simulink library "PacketizedNetworkLib"  (R2025b)
settings: Solver=VariableStepAuto  StartTime=0.0  StopTime=10.0  RelTol=1e-3
values from neighbouring files (symbols this model uses):
  dfeRef = [0.707106781187 -0.707106781187 0.707106781187 0.707106781187 -0.707106781187 0.707106781187 0.707106781187 0.707106781187 0.707106781187 0.707106781187 -0.707106781187 0.707106781187 ... (500 elements, 500x1)]    [networkParams.mat]
  L3payload = [0 0 0 1 0 0 0 0 1 1 1 0 ... (1040 elements, 1040x1)]    [networkParams.mat]
  ppdu_bb = [0 0 1 1 0 0 0 0 1 1 0 0 ... (2280 elements, 2280x1)]    [networkParams.mat]
  Ts = 1e-07    [networkParams.mat]
undefined symbols (not defined in the file or in its folder): AckDestAddre, DestAddre, dfilt, High, lambda, NodeAddre, pseed
libraries: $bdroot x19, hdlsllib x5, dspsigops x5, dspswit3 x3, simulink x3, dspindex x3, commdigbbndpm3 x2, simulink_extras x2, commfilt2 x2, commchan3 x1, dspmathops x1, dsparch4 x1
(part 2 of 3)

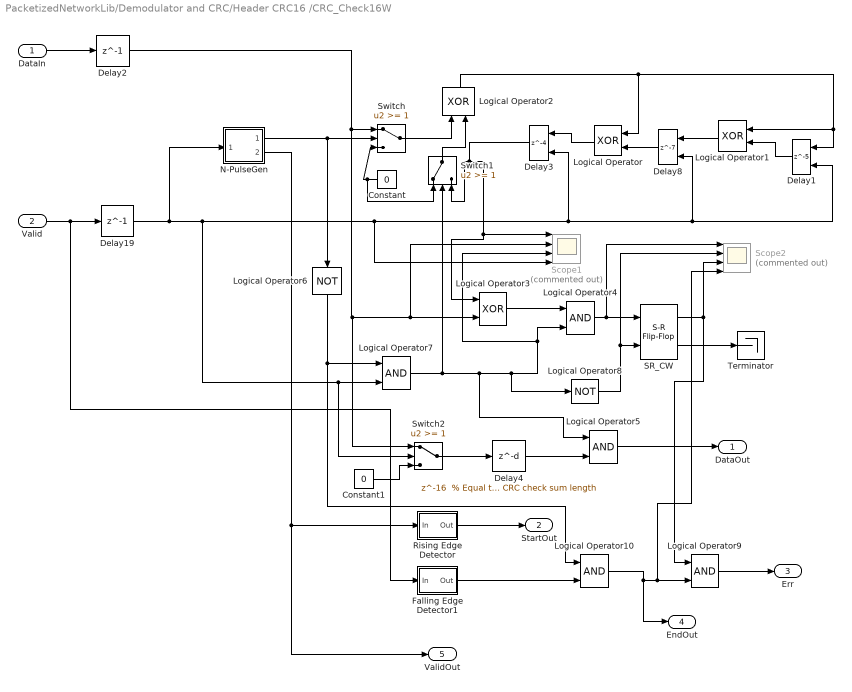
== system PacketizedNetworkLib/Demodulator and CRC/Header CRC16 /CRC_Check16W ==
  DataIn : Inport
  Valid : Inport  Port=2
  Constant : Constant  Value=0  OutDataTypeStr=boolean  SampleTime=-1
  Constant1 : Constant  Value=0  OutDataTypeStr=boolean  SampleTime=-1
  Delay1 : Delay  DelayLength=5  InitialCondition=0  ExternalReset=Rising
      settings: InputPortMap=u0,r5
  Delay19 : Delay  DelayLength=1
  Delay2 : Delay  DelayLength=1
  Delay3 : Delay  DelayLength=4  InitialCondition=0  ExternalReset=Rising
      settings: InputPortMap=u0,r5
  Delay4 : Delay  DelayLength="16  % Equal to the CRC check sum length"  InitialCondition=0
  Delay8 : Delay  DelayLength=7  InitialCondition=0  ExternalReset=Rising
      settings: InputPortMap=u0,r5
  Falling Edge Detector1 : Subsystem
  Logical Operator{,1..3} (4 alike) : Logic  Operator=XOR  AllPortsSameDT=off  OutDataTypeStr=boolean
  Logical Operator{4..5,7,9..10} (5 alike) : Logic  AllPortsSameDT=off  OutDataTypeStr=boolean
  Logical Operator6 : Logic  Operator=NOT  AllPortsSameDT=off  OutDataTypeStr=boolean
  Logical Operator8 : Logic  Operator=NOT  AllPortsSameDT=off  OutDataTypeStr=boolean
  N-PulseGen : Subsystem
  Rising Edge Detector : Subsystem
  SR_CW : simulink_extras/Flip Flops/S-R Flip-Flop  initial_condition=0
  Scope1 : Scope  Commented=on  NumInputPorts=4
      settings: ActiveDisplayYMinimum=-0.125  ActiveDisplayYMaximum=1.125  DataLoggingVariableName=ScopeData4  DataLoggingSaveFormat=Array
  Scope2 : Scope  Commented=on  NumInputPorts=4
      settings: ActiveDisplayYMinimum=-1  ActiveDisplayYMaximum=1  DataLoggingSaveFormat=Array
  Switch : Switch  Threshold=1  OutDataTypeStr=Inherit: Inherit via back propagation  SaturateOnIntegerOverflow=off
  Switch1 : Switch  Threshold=1  OutDataTypeStr=Inherit: Inherit via back propagation  SaturateOnIntegerOverflow=off
  Switch2 : Switch  Threshold=1  OutDataTypeStr=Inherit: Inherit via back propagation  SaturateOnIntegerOverflow=off
  Terminator : Terminator
  DataOut : Outport  VectorParamsAs1DForOutWhenUnconnected=off
  StartOut : Outport  Port=2  VectorParamsAs1DForOutWhenUnconnected=off
  Err : Outport  Port=3  VectorParamsAs1DForOutWhenUnconnected=off
  EndOut : Outport  Port=4  VectorParamsAs1DForOutWhenUnconnected=off
  ValidOut : Outport  Port=5  VectorParamsAs1DForOutWhenUnconnected=off
  wires:
  Logical Operator5/1 -> DataOut/1
  Logical Operator/1 -> Delay3/1
  Logical Operator10/1 -> Logical Operator9/2, Scope2/4, EndOut/1
  Delay19/1 -> N-PulseGen/1(In1), Switch2/2, Logical Operator7/2, Delay3/2, Delay1/2, Delay8/2, Scope1/4
  N-PulseGen/2(Out2) -> Rising Edge Detector/1(In), ValidOut/1
  Switch2/1 -> Delay4/1
  Constant1/1 -> Switch2/3
  Valid/1 -> Delay19/1, Falling Edge Detector1/1(In)
  Delay2/1 -> Logical Operator3/2, Scope1/2, Switch2/1, Switch/1
  Switch1/1 -> Logical Operator2/2
  Logical Operator6/1 -> Logical Operator7/1, Logical Operator10/1
  Delay1/1 -> Logical Operator1/2
  Logical Operator1/1 -> Delay8/1
  Delay8/1 -> Logical Operator/2
  Logical Operator8/1 -> Scope2/2, SR_CW/2
  Logical Operator7/1 -> Logical Operator4/2, Scope1/3, Logical Operator8/1, Logical Operator5/1, Switch1/2
  Logical Operator3/1 -> Logical Operator4/1
  N-PulseGen/1(Out1) -> Switch/2, Logical Operator6/1
  Logical Operator4/1 -> Scope2/1, SR_CW/1
  DataIn/1 -> Delay2/1
  Switch/1 -> Logical Operator2/1
  Delay3/1 -> Switch1/3, Scope1/1, Logical Operator3/1
  Constant/1 -> Switch/3, Switch1/1
  Logical Operator9/1 -> Err/1
  Falling Edge Detector1/1(Out) -> Logical Operator10/2
  SR_CW/1 -> Scope2/3, Logical Operator9/1
  Delay4/1 -> Logical Operator5/2
  Rising Edge Detector/1(Out) -> StartOut/1
  SR_CW/2 -> Terminator/1
  Logical Operator2/1 -> Logical Operator1/1, Delay1/1, Logical Operator/1

== system PacketizedNetworkLib/Demodulator and CRC/Pyld CRC32/Falling Edge Detector1 ==
  In : Inport
  Data Type Conversion2 : DataTypeConversion  OutDataTypeStr=boolean
  Delay : Delay  DelayLength=1  InitialCondition=1
  Logical Operator1 : Logic
  Logical Operator3 : Logic  Operator=NOT  Inputs=1
  Out : Outport  VectorParamsAs1DForOutWhenUnconnected=off
  wires:
  Logical Operator3/1 -> Logical Operator1/1
  Data Type Conversion2/1 -> Logical Operator3/1, Delay/1
  Delay/1 -> Logical Operator1/2
  In/1 -> Data Type Conversion2/1
  Logical Operator1/1 -> Out/1

== system PacketizedNetworkLib/Demodulator and CRC/Pyld CRC32/Rising Edge Detector ==
  In : Inport
  Data Type Conversion2 : DataTypeConversion  OutDataTypeStr=boolean
  Delay : Delay  DelayLength=1  InitialCondition=1
  Logical Operator : Logic  Operator=NOT  Inputs=1
  Logical Operator1 : Logic
  Out : Outport  VectorParamsAs1DForOutWhenUnconnected=off
  wires:
  Data Type Conversion2/1 -> Logical Operator1/1, Delay/1
  Logical Operator/1 -> Logical Operator1/2
  In/1 -> Data Type Conversion2/1
  Logical Operator1/1 -> Out/1
  Delay/1 -> Logical Operator/1

== system PacketizedNetworkLib/PHY//MAC Transceiver/Subsystem/BusSwitchFunIn ==
  Sel : Inport
  In1 : Inport  Port=2
  In2 : Inport  Port=3
  Bus Creator : BusCreator  Inputs=6
  Bus Selector1 : BusSelector  OutputSignals=TxDataFail,TxDataDone,TxDataOn,TxAckOn,BOTime,AckWaitTime
  Bus Selector2 : BusSelector  OutputSignals=TxDataFail,TxDataDone,TxDataOn,TxAckOn,BOTime,AckWaitTime
  Switch{,1..5} (6 alike) : Switch  Criteria=u2 > Threshold  SaturateOnIntegerOverflow=off  InputSameDT=off
  Out : Outport  VectorParamsAs1DForOutWhenUnconnected=off
  wires:
  Bus Creator/1 -> Out/1
  Switch5/1 -> Bus Creator/6
  Switch4/1 -> Bus Creator/5
  Switch3/1 -> Bus Creator/4
  Switch2/1 -> Bus Creator/3
  Switch1/1 -> Bus Creator/2
  Switch/1 -> Bus Creator/1
  In1/1 -> Bus Selector1/1
  Bus Selector1/6 -> Switch5/1  "<AckWaitTime>"
  Bus Selector1/5 -> Switch4/1  "<BOTime>"
  Bus Selector1/2 -> Switch1/1  "<TxDataDone>"
  Bus Selector1/1 -> Switch/1  "<TxDataFail>"
  Sel/1 -> Switch/2, Switch2/2, Switch5/2, Switch4/2, Switch3/2, Switch1/2
  Bus Selector1/3 -> Switch2/1  "<TxDataOn>"
  Bus Selector1/4 -> Switch3/1  "<TxAckOn>"
  Bus Selector2/1 -> Switch/3  "<TxDataFail>"
  Bus Selector2/2 -> Switch1/3  "<TxDataDone>"
  Bus Selector2/3 -> Switch2/3  "<TxDataOn>"
  Bus Selector2/4 -> Switch3/3  "<TxAckOn>"
  Bus Selector2/5 -> Switch4/3  "<BOTime>"
  Bus Selector2/6 -> Switch5/3  "<AckWaitTime>"
  In2/1 -> Bus Selector2/1

== system PacketizedNetworkLib/PHY//MAC Transceiver/Subsystem/BusSwitchFunOut ==
  Sel : Inport
  In : Inport  Port=2
  1to2_1 : Subsystem
  1to2_2 : Subsystem
  1to2_3 : Subsystem
  1to2_5 : Subsystem
  1to2_6 : Subsystem
  1to2_Integer : Subsystem
  Bus Creator1 : BusCreator  Inputs=6
  Bus Creator2 : BusCreator  Inputs=6
  Bus Selector1 : BusSelector  OutputSignals=TxLength,TxEn,signal3,signal4,signal5,signal6
  Out1 : Outport  VectorParamsAs1DForOutWhenUnconnected=off
  Out2 : Outport  Port=2  VectorParamsAs1DForOutWhenUnconnected=off
  wires:
  Bus Selector1/4 -> 1to2_3/1(In)  "<signal4>"
  Bus Selector1/3 -> 1to2_2/1(In)  "<signal3>"
  Bus Selector1/1 -> 1to2_Integer/1(In)  "<TxLength>"
  Bus Selector1/2 -> 1to2_1/1(In)  "<TxEn>"
  Bus Selector1/5 -> 1to2_5/1(In)  "<signal5>"
  Bus Selector1/6 -> 1to2_6/1(In)  "<signal6>"
  In/1 -> Bus Selector1/1
  Bus Creator2/1 -> Out1/1
  Bus Creator1/1 -> Out2/1
  Sel/1 -> 1to2_1/2(C), 1to2_2/2(C), 1to2_3/2(C), 1to2_6/2(C), 1to2_5/2(C), 1to2_Integer/2(C)
  1to2_Integer/1(Out1) -> Bus Creator2/1
  1to2_1/1(Out1) -> Bus Creator2/2
  1to2_2/1(Out1) -> Bus Creator2/3
  1to2_3/1(Out1) -> Bus Creator2/4
  1to2_5/1(Out1) -> Bus Creator2/5
  1to2_6/1(Out1) -> Bus Creator2/6
  1to2_Integer/2(Out2) -> Bus Creator1/1
  1to2_1/2(Out2) -> Bus Creator1/2
  1to2_2/2(Out2) -> Bus Creator1/3
  1to2_5/2(Out2) -> Bus Creator1/5
  1to2_3/2(Out2) -> Bus Creator1/4
  1to2_6/2(Out2) -> Bus Creator1/6

== system PacketizedNetworkLib/Receiver/DFE /DFE_Cell_FBW1 ==
  note: w(i)
  note: The Basic Cell of the Feedbackward Part of DFE Equalizer
      |
      | yd(i+1)= w(i+1).*d(i);
      | w(i+1)=w(i)+ m*D* w(i)=w(i)+etmu*conj(x(i));
      |
      | Note: All variables here are scalars
  note: w(i+1)
  d(i) : Inport
  etmu : Inport  Port=2
  " Unit_Delay1" : UnitDelay  SampleTime=-1  HasFrameUpgradeWarning=on
  " Unit_Delay2" : UnitDelay  SampleTime=-1  HasFrameUpgradeWarning=on
  Math Function : Math  Operator=conj  SignedPower=on
  Product1 : Product  InputSameDT=on  RndMeth=Zero  SaturateOnIntegerOverflow=on  OutDataTypeStr=Inherit: Same as first input
  Product2 : Product  InputSameDT=on  RndMeth=Zero  SaturateOnIntegerOverflow=on  OutDataTypeStr=Inherit: Same as first input
  Sum : Sum  InputSameDT=on  SaturateOnIntegerOverflow=on  OutDataTypeStr=Inherit: Same as first input
  "Unit_Delay1 " : UnitDelay  SampleTime=-1  HasFrameUpgradeWarning=on
  "d(i-1) " : Outport  VectorParamsAs1DForOutWhenUnconnected=off
  yd(i+1) : Outport  Port=2  VectorParamsAs1DForOutWhenUnconnected=off
  wires:
  " Unit_Delay1"/1 -> Product2/1
  Math Function/1 -> Product2/2
  d(i)/1 -> "Unit_Delay1 "/1, Product1/2
  etmu/1 -> " Unit_Delay1"/1
  "Unit_Delay1 "/1 -> "d(i-1) "/1, Math Function/1
  " Unit_Delay2"/1 -> Sum/1
  Sum/1 -> " Unit_Delay2"/1, Product1/1
  Product1/1 -> yd(i+1)/1
  Product2/1 -> Sum/2

== system PacketizedNetworkLib/Receiver/DFE /DFE_Cell_FBW2 ==
  note: w(i+1)
  note: The Basic Cell of the Feedbackward Part of DFE Equalizer
      |
      | yd(i+1)= w(i+1).*d(i);
      | w(i+1)=w(i)+ m*D* w(i)=w(i)+etmu*conj(x(i));
      |
      | Note: All variables here are scalars
  note: w(i)
  d(i) : Inport
  etmu : Inport  Port=2
  " Unit_Delay1" : UnitDelay  SampleTime=-1  HasFrameUpgradeWarning=on
  " Unit_Delay2" : UnitDelay  SampleTime=-1  HasFrameUpgradeWarning=on
  Math Function : Math  Operator=conj  SignedPower=on
  Product1 : Product  InputSameDT=on  RndMeth=Zero  SaturateOnIntegerOverflow=on  OutDataTypeStr=Inherit: Same as first input
  Product2 : Product  InputSameDT=on  RndMeth=Zero  SaturateOnIntegerOverflow=on  OutDataTypeStr=Inherit: Same as first input
  Sum : Sum  InputSameDT=on  SaturateOnIntegerOverflow=on  OutDataTypeStr=Inherit: Same as first input
  "Unit_Delay1 " : UnitDelay  SampleTime=-1  HasFrameUpgradeWarning=on
  "d(i-1) " : Outport  VectorParamsAs1DForOutWhenUnconnected=off
  yd(i+1) : Outport  Port=2  VectorParamsAs1DForOutWhenUnconnected=off
  wires:
  Product2/1 -> Sum/2
  Product1/1 -> yd(i+1)/1
  Sum/1 -> Product1/1, " Unit_Delay2"/1
  " Unit_Delay2"/1 -> Sum/1
  "Unit_Delay1 "/1 -> Math Function/1, "d(i-1) "/1
  etmu/1 -> " Unit_Delay1"/1
  d(i)/1 -> Product1/2, "Unit_Delay1 "/1
  Math Function/1 -> Product2/2
  " Unit_Delay1"/1 -> Product2/1

== system PacketizedNetworkLib/Receiver/DFE /DFE_Cell_FBW3 ==
  note: w(i+1)
  note: The Basic Cell of the Feedbackward Part of DFE Equalizer
      |
      | yd(i+1)= w(i+1).*d(i);
      | w(i+1)=w(i)+ m*D* w(i)=w(i)+etmu*conj(x(i));
      |
      | Note: All variables here are scalars
  note: w(i)
  d(i) : Inport
  etmu : Inport  Port=2
  " Unit_Delay1" : UnitDelay  SampleTime=-1  HasFrameUpgradeWarning=on
  " Unit_Delay2" : UnitDelay  SampleTime=-1  HasFrameUpgradeWarning=on
  Math Function : Math  Operator=conj  SignedPower=on
  Product1 : Product  InputSameDT=on  RndMeth=Zero  SaturateOnIntegerOverflow=on  OutDataTypeStr=Inherit: Same as first input
  Product2 : Product  InputSameDT=on  RndMeth=Zero  SaturateOnIntegerOverflow=on  OutDataTypeStr=Inherit: Same as first input
  Sum : Sum  InputSameDT=on  SaturateOnIntegerOverflow=on  OutDataTypeStr=Inherit: Same as first input
  "Unit_Delay1 " : UnitDelay  SampleTime=-1  HasFrameUpgradeWarning=on
  "d(i-1) " : Outport  VectorParamsAs1DForOutWhenUnconnected=off
  yd(i+1) : Outport  Port=2  VectorParamsAs1DForOutWhenUnconnected=off
  wires:
  Product2/1 -> Sum/2
  Product1/1 -> yd(i+1)/1
  Sum/1 -> " Unit_Delay2"/1, Product1/1
  " Unit_Delay2"/1 -> Sum/1
  "Unit_Delay1 "/1 -> Math Function/1, "d(i-1) "/1
  etmu/1 -> " Unit_Delay1"/1
  d(i)/1 -> Product1/2, "Unit_Delay1 "/1
  Math Function/1 -> Product2/2
  " Unit_Delay1"/1 -> Product2/1

== system PacketizedNetworkLib/Receiver/DFE /DFE_Cell_FBW4 ==
  note: w(i+1)
  note: The Basic Cell of the Feedbackward Part of DFE Equalizer
      |
      | yd(i+1)= w(i+1).*d(i);
      | w(i+1)=w(i)+ m*D* w(i)=w(i)+etmu*conj(x(i));
  note: w(i)
  note: DFE Equalizer
  d(i) : Inport
  etmu : Inport  Port=2
  " Unit_Delay1" : UnitDelay  SampleTime=-1  HasFrameUpgradeWarning=on
  " Unit_Delay2" : UnitDelay  SampleTime=-1  HasFrameUpgradeWarning=on
  Math Function : Math  Operator=conj  SignedPower=on
  Product1 : Product  InputSameDT=on  RndMeth=Zero  SaturateOnIntegerOverflow=on  OutDataTypeStr=Inherit: Same as first input
  Product2 : Product  InputSameDT=on  RndMeth=Zero  SaturateOnIntegerOverflow=on  OutDataTypeStr=Inherit: Same as first input
  Sum : Sum  InputSameDT=on  SaturateOnIntegerOverflow=on  OutDataTypeStr=Inherit: Same as first input
  "Unit_Delay1 " : UnitDelay  SampleTime=-1  HasFrameUpgradeWarning=on
  "d(i-1) " : Outport  VectorParamsAs1DForOutWhenUnconnected=off
  yd(i+1) : Outport  Port=2  VectorParamsAs1DForOutWhenUnconnected=off
  wires:
  Product2/1 -> Sum/2
  Product1/1 -> yd(i+1)/1
  Sum/1 -> " Unit_Delay2"/1, Product1/1
  " Unit_Delay2"/1 -> Sum/1
  "Unit_Delay1 "/1 -> "d(i-1) "/1, Math Function/1
  etmu/1 -> " Unit_Delay1"/1
  d(i)/1 -> Product1/2, "Unit_Delay1 "/1
  Math Function/1 -> Product2/2
  " Unit_Delay1"/1 -> Product2/1

== system PacketizedNetworkLib/Receiver/DFE /DFE_Cell_FBW5 ==
  note: w(i+1)
  note: The Basic Cell of the Feedbackward Part of DFE Equalizer
      |
      | yd(i+1)= w(i+1).*d(i);
      | w(i+1)=w(i)+ m*D* w(i)=w(i)+etmu*conj(x(i));
      |
      | Note: All variables here are scalars
  note: w(i)
  d(i) : Inport
  etmu : Inport  Port=2
  " Unit_Delay1" : UnitDelay  SampleTime=-1  HasFrameUpgradeWarning=on
  " Unit_Delay2" : UnitDelay  SampleTime=-1  HasFrameUpgradeWarning=on
  Math Function : Math  Operator=conj  SignedPower=on
  Product1 : Product  InputSameDT=on  RndMeth=Zero  SaturateOnIntegerOverflow=on  OutDataTypeStr=Inherit: Same as first input
  Product2 : Product  InputSameDT=on  RndMeth=Zero  SaturateOnIntegerOverflow=on  OutDataTypeStr=Inherit: Same as first input
  Sum : Sum  InputSameDT=on  SaturateOnIntegerOverflow=on  OutDataTypeStr=Inherit: Same as first input
  "Unit_Delay1 " : UnitDelay  SampleTime=-1  HasFrameUpgradeWarning=on
  "d(i-1) " : Outport  VectorParamsAs1DForOutWhenUnconnected=off
  yd(i+1) : Outport  Port=2  VectorParamsAs1DForOutWhenUnconnected=off
  wires:
  Product2/1 -> Sum/2
  Product1/1 -> yd(i+1)/1
  Sum/1 -> " Unit_Delay2"/1, Product1/1
  " Unit_Delay2"/1 -> Sum/1
  "Unit_Delay1 "/1 -> Math Function/1, "d(i-1) "/1
  etmu/1 -> " Unit_Delay1"/1
  d(i)/1 -> Product1/2, "Unit_Delay1 "/1
  Math Function/1 -> Product2/2
  " Unit_Delay1"/1 -> Product2/1

== system PacketizedNetworkLib/Receiver/DFE /DFE_Cell_FBW6 ==
  note: w(i+1)
  note: The Basic Cell of the Feedbackward Part of DFE Equalizer
      |
      | yd(i+1)= w(i+1).*d(i);
      | w(i+1)=w(i)+ m*D* w(i)=w(i)+etmu*conj(x(i));
      |
      | Note: All variables here are scalars
  note: w(i)
  d(i) : Inport
  etmu : Inport  Port=2
  " Unit_Delay1" : UnitDelay  SampleTime=-1  HasFrameUpgradeWarning=on
  " Unit_Delay2" : UnitDelay  SampleTime=-1  HasFrameUpgradeWarning=on
  Math Function : Math  Operator=conj  SignedPower=on
  Product1 : Product  InputSameDT=on  RndMeth=Zero  SaturateOnIntegerOverflow=on  OutDataTypeStr=Inherit: Same as first input
  Product2 : Product  InputSameDT=on  RndMeth=Zero  SaturateOnIntegerOverflow=on  OutDataTypeStr=Inherit: Same as first input
  Sum : Sum  InputSameDT=on  SaturateOnIntegerOverflow=on  OutDataTypeStr=Inherit: Same as first input
  "Unit_Delay1 " : UnitDelay  SampleTime=-1  HasFrameUpgradeWarning=on
  "d(i-1) " : Outport  VectorParamsAs1DForOutWhenUnconnected=off
  yd(i+1) : Outport  Port=2  VectorParamsAs1DForOutWhenUnconnected=off
  wires:
  Product2/1 -> Sum/2
  Product1/1 -> yd(i+1)/1
  Sum/1 -> Product1/1, " Unit_Delay2"/1
  " Unit_Delay2"/1 -> Sum/1
  "Unit_Delay1 "/1 -> "d(i-1) "/1, Math Function/1
  etmu/1 -> " Unit_Delay1"/1
  d(i)/1 -> Product1/2, "Unit_Delay1 "/1
  Math Function/1 -> Product2/2
  " Unit_Delay1"/1 -> Product2/1

== system PacketizedNetworkLib/Receiver/DFE /DFE_Cell_FFW1 ==
  note: w(i+1)
  note: The Basic Cell of the Feedforward Part of DFE Equalizer
      |
      | y(i+1)= ElimentSum (w(i+1).*x(i+1));
      | w(i+1)=w(i)+ m*D* w(i)=w(i)+etmu*conj(x(i));
      |
      | Note: y(+1) and etmu is a scalar, and x(i), w(i) are 2x1 vector. "2" is the decimation factor 2
  note: w(i)
  x(i+1) : Inport
  etmu : Inport  Port=2
  " Unit_Delay1" : UnitDelay  SampleTime=-1  HasFrameUpgradeWarning=on
  " Unit_Delay2" : UnitDelay  SampleTime=-1  HasFrameUpgradeWarning=on
  Math Function : Math  Operator=conj  SignedPower=on
  Product1 : Product  InputSameDT=on  RndMeth=Zero  SaturateOnIntegerOverflow=on  OutDataTypeStr=Inherit: Same as first input
  Product2 : Product  InputSameDT=on  RndMeth=Zero  SaturateOnIntegerOverflow=on  OutDataTypeStr=Inherit: Same as first input
  Sum : Sum  InputSameDT=on  SaturateOnIntegerOverflow=on  OutDataTypeStr=Inherit: Same as first input
  Sum of Elements : Sum  Inputs=+
  "Unit_Delay1 " : UnitDelay  SampleTime=-1  HasFrameUpgradeWarning=on
  "x(i) " : Outport  VectorParamsAs1DForOutWhenUnconnected=off
  y(i+1) : Outport  Port=2  VectorParamsAs1DForOutWhenUnconnected=off
  wires:
  Product2/1 -> Sum/2
  Product1/1 -> Sum of Elements/1
  " Unit_Delay2"/1 -> Sum/1
  "Unit_Delay1 "/1 -> Math Function/1, "x(i) "/1
  etmu/1 -> " Unit_Delay1"/1
  x(i+1)/1 -> Product1/2, "Unit_Delay1 "/1
  Math Function/1 -> Product2/2
  Sum of Elements/1 -> y(i+1)/1
  Sum/1 -> Product1/1, " Unit_Delay2"/1
  " Unit_Delay1"/1 -> Product2/1

== system PacketizedNetworkLib/Receiver/DFE /DFE_Cell_FFW2 ==
  note: w(i+1)
  note: The Basic Cell of the Feedforward Part of DFE Equalizer
      |
      | y(i+1)= ElimentSum (w(i+1).*x(i+1));
      | w(i+1)=w(i)+ m*D* w(i)=w(i)+etmu*conj(x(i));
      |
      | Note: y(+1) and etmu is a scalar, and x(i), w(i) are 2x1 vector. "2" is the decimation factor 2
  note: w(i)
  x(i+1) : Inport
  etmu : Inport  Port=2
  " Unit_Delay1" : UnitDelay  SampleTime=-1  HasFrameUpgradeWarning=on
  " Unit_Delay2" : UnitDelay  SampleTime=-1  HasFrameUpgradeWarning=on
  Math Function : Math  Operator=conj  SignedPower=on
  Product1 : Product  InputSameDT=on  RndMeth=Zero  SaturateOnIntegerOverflow=on  OutDataTypeStr=Inherit: Same as first input
  Product2 : Product  InputSameDT=on  RndMeth=Zero  SaturateOnIntegerOverflow=on  OutDataTypeStr=Inherit: Same as first input
  Sum : Sum  InputSameDT=on  SaturateOnIntegerOverflow=on  OutDataTypeStr=Inherit: Same as first input
  Sum of Elements : Sum  Inputs=+
  "Unit_Delay1 " : UnitDelay  SampleTime=-1  HasFrameUpgradeWarning=on
  "x(i) " : Outport  VectorParamsAs1DForOutWhenUnconnected=off
  y(i+1) : Outport  Port=2  VectorParamsAs1DForOutWhenUnconnected=off
  wires:
  Product2/1 -> Sum/2
  Product1/1 -> Sum of Elements/1
  " Unit_Delay2"/1 -> Sum/1
  "Unit_Delay1 "/1 -> Math Function/1, "x(i) "/1
  etmu/1 -> " Unit_Delay1"/1
  x(i+1)/1 -> Product1/2, "Unit_Delay1 "/1
  Math Function/1 -> Product2/2
  Sum of Elements/1 -> y(i+1)/1
  Sum/1 -> Product1/1, " Unit_Delay2"/1
  " Unit_Delay1"/1 -> Product2/1

== system PacketizedNetworkLib/Receiver/DFE /DFE_Cell_FFW3 ==
  note: w(i+1)
  note: The Basic Cell of the Feedforward Part of DFE Equalizer
      |
      | y(i+1)= ElimentSum (w(i+1).*x(i+1));
      | w(i+1)=w(i)+ m*D* w(i)=w(i)+etmu*conj(x(i));
      |
      | Note: y(+1) and etmu is a scalar, and x(i), w(i) are 2x1 vector. "2" is the decimation factor 2
  note: w(i)
  x(i+1) : Inport
  etmu : Inport  Port=2
  " Unit_Delay1" : UnitDelay  SampleTime=-1  HasFrameUpgradeWarning=on
  " Unit_Delay2" : UnitDelay  SampleTime=-1  HasFrameUpgradeWarning=on
  Math Function : Math  Operator=conj  SignedPower=on
  Product1 : Product  InputSameDT=on  RndMeth=Zero  SaturateOnIntegerOverflow=on  OutDataTypeStr=Inherit: Same as first input
  Product2 : Product  InputSameDT=on  RndMeth=Zero  SaturateOnIntegerOverflow=on  OutDataTypeStr=Inherit: Same as first input
  Sum : Sum  InputSameDT=on  SaturateOnIntegerOverflow=on  OutDataTypeStr=Inherit: Same as first input
  Sum of Elements : Sum  Inputs=+
  "Unit_Delay1 " : UnitDelay  SampleTime=-1  HasFrameUpgradeWarning=on
  "x(i) " : Outport  VectorParamsAs1DForOutWhenUnconnected=off
  y(i+1) : Outport  Port=2  VectorParamsAs1DForOutWhenUnconnected=off
  wires:
  Product2/1 -> Sum/2
  Product1/1 -> Sum of Elements/1
  " Unit_Delay2"/1 -> Sum/1
  "Unit_Delay1 "/1 -> Math Function/1, "x(i) "/1
  etmu/1 -> " Unit_Delay1"/1
  x(i+1)/1 -> Product1/2, "Unit_Delay1 "/1
  Math Function/1 -> Product2/2
  Sum of Elements/1 -> y(i+1)/1
  Sum/1 -> Product1/1, " Unit_Delay2"/1
  " Unit_Delay1"/1 -> Product2/1

== system PacketizedNetworkLib/Receiver/DFE /DFE_Cell_FFW4 ==
  note: w(i+1)
  note: The Basic Cell of the Feedforward Part of DFE Equalizer
      |
      | y(i+1)= ElimentSum (w(i+1).*x(i+1));
      | w(i+1)=w(i)+ m*D* w(i)=w(i)+etmu*conj(x(i));
      |
      | Note: y(+1) and etmu is a scalar, and x(i), w(i) are 2x1 vector. "2" is the decimation factor 2
  note: w(i)
  x(i+1) : Inport
  etmu : Inport  Port=2
  " Unit_Delay1" : UnitDelay  SampleTime=-1  HasFrameUpgradeWarning=on
  " Unit_Delay2" : UnitDelay  SampleTime=-1  HasFrameUpgradeWarning=on
  Math Function : Math  Operator=conj  SignedPower=on
  Product1 : Product  InputSameDT=on  RndMeth=Zero  SaturateOnIntegerOverflow=on  OutDataTypeStr=Inherit: Same as first input
  Product2 : Product  InputSameDT=on  RndMeth=Zero  SaturateOnIntegerOverflow=on  OutDataTypeStr=Inherit: Same as first input
  Sum : Sum  InputSameDT=on  SaturateOnIntegerOverflow=on  OutDataTypeStr=Inherit: Same as first input
  Sum of Elements : Sum  Inputs=+
  "Unit_Delay1 " : UnitDelay  SampleTime=-1  HasFrameUpgradeWarning=on
  "x(i) " : Outport  VectorParamsAs1DForOutWhenUnconnected=off
  y(i+1) : Outport  Port=2  VectorParamsAs1DForOutWhenUnconnected=off
  wires:
  Product2/1 -> Sum/2
  Product1/1 -> Sum of Elements/1
  " Unit_Delay2"/1 -> Sum/1
  "Unit_Delay1 "/1 -> Math Function/1, "x(i) "/1
  etmu/1 -> " Unit_Delay1"/1
  x(i+1)/1 -> Product1/2, "Unit_Delay1 "/1
  Math Function/1 -> Product2/2
  Sum of Elements/1 -> y(i+1)/1
  Sum/1 -> Product1/1, " Unit_Delay2"/1
  " Unit_Delay1"/1 -> Product2/1

== system PacketizedNetworkLib/Receiver/DFE /DFE_Cell_FFW5 ==
  note: w(i+1)
  note: The Basic Cell of the Feedforward Part of DFE Equalizer
      |
      | y(i+1)= ElimentSum (w(i+1).*x(i+1));
      | w(i+1)=w(i)+ m*D* w(i)=w(i)+etmu*conj(x(i));
      |
      | Note: y(+1) and etmu is a scalar, and x(i), w(i) are 2x1 vector. "2" is the decimation factor 2
  note: w(i)
  x(i+1) : Inport
  etmu : Inport  Port=2
  " Unit_Delay1" : UnitDelay  SampleTime=-1  HasFrameUpgradeWarning=on
  " Unit_Delay2" : UnitDelay  SampleTime=-1  HasFrameUpgradeWarning=on
  Math Function : Math  Operator=conj  SignedPower=on
  Product1 : Product  InputSameDT=on  RndMeth=Zero  SaturateOnIntegerOverflow=on  OutDataTypeStr=Inherit: Same as first input
  Product2 : Product  InputSameDT=on  RndMeth=Zero  SaturateOnIntegerOverflow=on  OutDataTypeStr=Inherit: Same as first input
  Sum : Sum  InputSameDT=on  SaturateOnIntegerOverflow=on  OutDataTypeStr=Inherit: Same as first input
  Sum of Elements : Sum  Inputs=+
  "Unit_Delay1 " : UnitDelay  SampleTime=-1  HasFrameUpgradeWarning=on
  "x(i) " : Outport  VectorParamsAs1DForOutWhenUnconnected=off
  y(i+1) : Outport  Port=2  VectorParamsAs1DForOutWhenUnconnected=off
  wires:
  Product2/1 -> Sum/2
  Product1/1 -> Sum of Elements/1
  " Unit_Delay2"/1 -> Sum/1
  "Unit_Delay1 "/1 -> Math Function/1, "x(i) "/1
  etmu/1 -> " Unit_Delay1"/1
  x(i+1)/1 -> Product1/2, "Unit_Delay1 "/1
  Math Function/1 -> Product2/2
  Sum of Elements/1 -> y(i+1)/1
  Sum/1 -> Product1/1, " Unit_Delay2"/1
  " Unit_Delay1"/1 -> Product2/1

== system PacketizedNetworkLib/Receiver/DFE /DFE_Cell_FFW6 ==
  note: w(i+1)
  note: The Basic Cell of the Feedforward Part of DFE Equalizer
      |
      | y(i+1)= ElimentSum (w(i+1).*x(i+1));
      | w(i+1)=w(i)+ m*D* w(i)=w(i)+etmu*conj(x(i));
      |
      | Note: y(+1) and etmu is a scalar, and x(i), w(i) are 2x1 vector. "2" is the decimation factor 2
  note: w(i)
  x(i+1) : Inport
  etmu : Inport  Port=2
  " Unit_Delay1" : UnitDelay  SampleTime=-1  HasFrameUpgradeWarning=on
  " Unit_Delay2" : UnitDelay  SampleTime=-1  HasFrameUpgradeWarning=on
  Math Function : Math  Operator=conj  SignedPower=on
  Product1 : Product  InputSameDT=on  RndMeth=Zero  SaturateOnIntegerOverflow=on  OutDataTypeStr=Inherit: Same as first input
  Product2 : Product  InputSameDT=on  RndMeth=Zero  SaturateOnIntegerOverflow=on  OutDataTypeStr=Inherit: Same as first input
  Sum : Sum  InputSameDT=on  SaturateOnIntegerOverflow=on  OutDataTypeStr=Inherit: Same as first input
  Sum of Elements : Sum  Inputs=+
  "Unit_Delay1 " : UnitDelay  SampleTime=-1  HasFrameUpgradeWarning=on
  "x(i) " : Outport  VectorParamsAs1DForOutWhenUnconnected=off
  y(i+1) : Outport  Port=2  VectorParamsAs1DForOutWhenUnconnected=off
  wires:
  Product2/1 -> Sum/2
  Product1/1 -> Sum of Elements/1
  " Unit_Delay2"/1 -> Sum/1
  "Unit_Delay1 "/1 -> Math Function/1, "x(i) "/1
  etmu/1 -> " Unit_Delay1"/1
  x(i+1)/1 -> Product1/2, "Unit_Delay1 "/1
  Math Function/1 -> Product2/2
  Sum of Elements/1 -> y(i+1)/1
  Sum/1 -> Product1/1, " Unit_Delay2"/1
  " Unit_Delay1"/1 -> Product2/1

== system PacketizedNetworkLib/Receiver/DFE /DFE_Cell_FFW7 ==
  note: w(i+1)
  note: The Basic Cell of the Feedforward Part of DFE Equalizer
      |
      | y(i+1)= ElimentSum (w(i+1).*x(i+1));
      | w(i+1)=w(i)+ m*D* w(i)=w(i)+etmu*conj(x(i));
      |
      | Note: y(+1) and etmu is a scalar, and x(i), w(i) are 2x1 vector. "2" is the decimation factor 2
  note: w(i)
  x(i+1) : Inport
  etmu : Inport  Port=2
  " Unit_Delay1" : UnitDelay  SampleTime=-1  HasFrameUpgradeWarning=on
  " Unit_Delay2" : UnitDelay  SampleTime=-1  HasFrameUpgradeWarning=on
  Math Function : Math  Operator=conj  SignedPower=on
  Product1 : Product  InputSameDT=on  RndMeth=Zero  SaturateOnIntegerOverflow=on  OutDataTypeStr=Inherit: Same as first input
  Product2 : Product  InputSameDT=on  RndMeth=Zero  SaturateOnIntegerOverflow=on  OutDataTypeStr=Inherit: Same as first input
  Sum : Sum  InputSameDT=on  SaturateOnIntegerOverflow=on  OutDataTypeStr=Inherit: Same as first input
  Sum of Elements : Sum  Inputs=+
  "Unit_Delay1 " : UnitDelay  SampleTime=-1  HasFrameUpgradeWarning=on
  "x(i) " : Outport  VectorParamsAs1DForOutWhenUnconnected=off
  y(i+1) : Outport  Port=2  VectorParamsAs1DForOutWhenUnconnected=off
  wires:
  Product2/1 -> Sum/2
  Product1/1 -> Sum of Elements/1
  " Unit_Delay2"/1 -> Sum/1
  "Unit_Delay1 "/1 -> Math Function/1, "x(i) "/1
  etmu/1 -> " Unit_Delay1"/1
  x(i+1)/1 -> Product1/2, "Unit_Delay1 "/1
  Math Function/1 -> Product2/2
  Sum of Elements/1 -> y(i+1)/1
  Sum/1 -> Product1/1, " Unit_Delay2"/1
  " Unit_Delay1"/1 -> Product2/1

== system PacketizedNetworkLib/Receiver/DFE /DFE_Cell_FFW8 ==
  note: w(i+1)
  note: The Basic Cell of the Feedforward Part of DFE Equalizer
      |
      | y(i+1)= ElimentSum (w(i+1).*x(i+1));
      | w(i+1)=w(i)+ m*D* w(i)=w(i)+etmu*conj(x(i));
      |
      | Note: y(+1) and etmu is a scalar, and x(i), w(i) are 2x1 vector. "2" is the decimation factor 2
  note: w(i)
  x(i+1) : Inport
  etmu : Inport  Port=2
  " Unit_Delay1" : UnitDelay  SampleTime=-1  HasFrameUpgradeWarning=on
  " Unit_Delay2" : UnitDelay  SampleTime=-1  HasFrameUpgradeWarning=on
  Math Function : Math  Operator=conj  SignedPower=on
  Product1 : Product  InputSameDT=on  RndMeth=Zero  SaturateOnIntegerOverflow=on  OutDataTypeStr=Inherit: Same as first input
  Product2 : Product  InputSameDT=on  RndMeth=Zero  SaturateOnIntegerOverflow=on  OutDataTypeStr=Inherit: Same as first input
  Sum : Sum  InputSameDT=on  SaturateOnIntegerOverflow=on  OutDataTypeStr=Inherit: Same as first input
  Sum of Elements : Sum  Inputs=+
  "Unit_Delay1 " : UnitDelay  SampleTime=-1  HasFrameUpgradeWarning=on
  "x(i) " : Outport  VectorParamsAs1DForOutWhenUnconnected=off
  y(i+1) : Outport  Port=2  VectorParamsAs1DForOutWhenUnconnected=off
  wires:
  Product2/1 -> Sum/2
  Product1/1 -> Sum of Elements/1
  " Unit_Delay2"/1 -> Sum/1
  "Unit_Delay1 "/1 -> Math Function/1, "x(i) "/1
  etmu/1 -> " Unit_Delay1"/1
  x(i+1)/1 -> Product1/2, "Unit_Delay1 "/1
  Math Function/1 -> Product2/2
  Sum of Elements/1 -> y(i+1)/1
  Sum/1 -> Product1/1, " Unit_Delay2"/1
  " Unit_Delay1"/1 -> Product2/1

== system PacketizedNetworkLib/Receiver/DFE /DFE_Cell_FFW9 ==
  note: w(i+1)
  note: The Basic Cell of the Feedforward Part of DFE Equalizer
      |
      | y(i+1)= ElimentSum (w(i+1).*x(i+1));
      | w(i+1)=w(i)+ m*D* w(i)=w(i)+etmu*conj(x(i));
      |
      | Note: y(+1) and etmu is a scalar, and x(i), w(i) are 2x1 vector. "2" is the decimation factor 2
  note: w(i)
  x(i+1) : Inport
  etmu : Inport  Port=2
  " Unit_Delay1" : UnitDelay  SampleTime=-1  HasFrameUpgradeWarning=on
  " Unit_Delay2" : UnitDelay  SampleTime=-1  HasFrameUpgradeWarning=on
  Math Function : Math  Operator=conj  SignedPower=on
  Product1 : Product  InputSameDT=on  RndMeth=Zero  SaturateOnIntegerOverflow=on  OutDataTypeStr=Inherit: Same as first input
  Product2 : Product  InputSameDT=on  RndMeth=Zero  SaturateOnIntegerOverflow=on  OutDataTypeStr=Inherit: Same as first input
  Sum : Sum  InputSameDT=on  SaturateOnIntegerOverflow=on  OutDataTypeStr=Inherit: Same as first input
  Sum of Elements : Sum  Inputs=+
  "Unit_Delay1 " : UnitDelay  SampleTime=-1  HasFrameUpgradeWarning=on
  "x(i) " : Outport  VectorParamsAs1DForOutWhenUnconnected=off
  y(i+1) : Outport  Port=2  VectorParamsAs1DForOutWhenUnconnected=off
  wires:
  Product2/1 -> Sum/2
  Product1/1 -> Sum of Elements/1
  " Unit_Delay2"/1 -> Sum/1
  "Unit_Delay1 "/1 -> Math Function/1, "x(i) "/1
  etmu/1 -> " Unit_Delay1"/1
  x(i+1)/1 -> Product1/2, "Unit_Delay1 "/1
  Math Function/1 -> Product2/2
  Sum of Elements/1 -> y(i+1)/1
  Sum/1 -> Product1/1, " Unit_Delay2"/1
  " Unit_Delay1"/1 -> Product2/1

== system PacketizedNetworkLib/Receiver/Signal Detection/Signal Detect ==
  In1 : Inport
  Biquad Filter : dsparch4/Biquad Filter  Commented=on  FilterSource=Dialog parameters  CoeffSource=Specify via dialog  FilterObject=dfilt.df2tsos([1 0.3 0.4],[1 0.1 0.2])  IIRFiltStruct=Direct form II transposed  BiQuadCoeffs=[0.01 0 0 1 -1.8 0.81]  ScaleValues=1  IC=0  ICnum=0  ICden=0  a0Flag=Warning  optimizeScaleValues=on  ScaleValueMode=Specify via input port (g)  roundingMode=Floor  overflowMode=off  scaleValueFracLength=14  denProdOutputFracLength=30  denAccumFracLength=30  secondMemoryFracLength=15
  Gain : Gain  Gain=0.9
  Gain1 : Gain  Gain=0.9
  Sum : Sum  Inputs=|-+
  Sum1 : Sum  Inputs=|++
  Sum2 : Sum  Inputs=|-+
  Sum3 : Sum  Inputs=|++
  Unit Delay : UnitDelay  SampleTime=-1  HasFrameUpgradeWarning=on
  Unit Delay1 : UnitDelay  SampleTime=-1  HasFrameUpgradeWarning=on
  Out1 : Outport  VectorParamsAs1DForOutWhenUnconnected=off
  wires:
  Gain/1 -> Sum1/2
  Unit Delay1/1 -> Sum2/2
  Sum3/1 -> Unit Delay1/1, Out1/1
  Gain1/1 -> Sum3/2
  Sum2/1 -> Gain1/1
  Sum1/1 -> Unit Delay/1, Sum2/1, Sum3/1
  In1/1 -> Sum/1, Sum1/1
  Sum/1 -> Gain/1
  Unit Delay/1 -> Sum/2

== system PacketizedNetworkLib/Demodulator and CRC/Header CRC16 /CRC_Check16W/Falling Edge Detector1 ==
  In : Inport
  Data Type Conversion2 : DataTypeConversion  OutDataTypeStr=boolean
  Delay : Delay  DelayLength=1  InitialCondition=1
  Logical Operator1 : Logic
  Logical Operator3 : Logic  Operator=NOT  Inputs=1
  Out : Outport  VectorParamsAs1DForOutWhenUnconnected=off
  wires:
  Logical Operator3/1 -> Logical Operator1/1
  Data Type Conversion2/1 -> Logical Operator3/1, Delay/1
  Delay/1 -> Logical Operator1/2
  In/1 -> Data Type Conversion2/1
  Logical Operator1/1 -> Out/1

== system PacketizedNetworkLib/Demodulator and CRC/Header CRC16 /CRC_Check16W/N-PulseGen ==
  In1 : Inport  OutDataTypeStr=boolean
  Compare To Constant : simulink/Logic and Bit Operations/Compare To Constant  relop=<=  const=16 %The length of data  OutDataTypeStr=boolean
  Compare To Constant1 : simulink/Logic and Bit Operations/Compare To Constant  relop=<=  const="16  % The length of check sum"  OutDataTypeStr=boolean
  HDL Counter3 : hdlsllib/Sources/HDL Counter  CountType=Count limited  CountInit=1  CountStep=1  CountMax=32 % The length of data + check sum  CountFromType=Initial value  CountFrom=1  CountResetPort=on  CountLoadPort=off  CountEnbPort=on  CountDirPort=off  CountHitOutputPort=off  CountDataType=Unsigned  CountWordLen=8  CountFracLen=0  CountSampTime=1
  Logical Operator : Logic  Operator=NOT  AllPortsSameDT=off  OutDataTypeStr=boolean
  Logical Operator2 : Logic  Operator=NOT  AllPortsSameDT=off  OutDataTypeStr=boolean
  Scope : Scope  NumInputPorts=4
      settings: ActiveDisplayYMinimum=-0.125  ActiveDisplayYMaximum=1.125  DataLoggingVariableName=ScopeData3
  Out1 : Outport  VectorParamsAs1DForOutWhenUnconnected=off
  Out2 : Outport  Port=2  VectorParamsAs1DForOutWhenUnconnected=off
  wires:
  Logical Operator2/1 -> Out2/1
  Compare To Constant1/1 -> Logical Operator2/1
  In1/1 -> Logical Operator/1, HDL Counter3/2, Scope/1
  Logical Operator/1 -> HDL Counter3/1
  Compare To Constant/1 -> Scope/3, Scope/4, Out1/1
  HDL Counter3/1 -> Compare To Constant/1, Compare To Constant1/1, Scope/2

== system PacketizedNetworkLib/Demodulator and CRC/Header CRC16 /CRC_Check16W/Rising Edge Detector ==
  In : Inport
  Data Type Conversion2 : DataTypeConversion  OutDataTypeStr=boolean
  Delay : Delay  DelayLength=1  InitialCondition=1
  Logical Operator : Logic  Operator=NOT  Inputs=1
  Logical Operator1 : Logic
  Out : Outport  VectorParamsAs1DForOutWhenUnconnected=off
  wires:
  Data Type Conversion2/1 -> Logical Operator1/1, Delay/1
  Logical Operator/1 -> Logical Operator1/2
  In/1 -> Data Type Conversion2/1
  Logical Operator1/1 -> Out/1
  Delay/1 -> Logical Operator/1

== system PacketizedNetworkLib/PHY//MAC Transceiver/Subsystem/BusSwitchFunOut/1to2_1 ==
  In : Inport
  C : Inport  Port=2
  Logical Operator1 : Logic  AllPortsSameDT=off  OutDataTypeStr=boolean
  Logical Operator2 : Logic  AllPortsSameDT=off  OutDataTypeStr=boolean
  Logical Operator3 : Logic  Operator=NOT  AllPortsSameDT=off  OutDataTypeStr=boolean
  Out1 : Outport  VectorParamsAs1DForOutWhenUnconnected=off
  Out2 : Outport  Port=2  VectorParamsAs1DForOutWhenUnconnected=off
  wires:
  Logical Operator2/1 -> Out2/1
  C/1 -> Logical Operator1/2, Logical Operator3/1
  In/1 -> Logical Operator2/1, Logical Operator1/1
  Logical Operator1/1 -> Out1/1
  Logical Operator3/1 -> Logical Operator2/2

== system PacketizedNetworkLib/PHY//MAC Transceiver/Subsystem/BusSwitchFunOut/1to2_2 ==
  In : Inport
  C : Inport  Port=2
  Logical Operator1 : Logic  AllPortsSameDT=off  OutDataTypeStr=boolean
  Logical Operator2 : Logic  AllPortsSameDT=off  OutDataTypeStr=boolean
  Logical Operator3 : Logic  Operator=NOT  AllPortsSameDT=off  OutDataTypeStr=boolean
  Out1 : Outport  VectorParamsAs1DForOutWhenUnconnected=off
  Out2 : Outport  Port=2  VectorParamsAs1DForOutWhenUnconnected=off
  wires:
  Logical Operator3/1 -> Logical Operator2/2
  Logical Operator1/1 -> Out1/1
  In/1 -> Logical Operator1/1, Logical Operator2/1
  C/1 -> Logical Operator3/1, Logical Operator1/2
  Logical Operator2/1 -> Out2/1

== system PacketizedNetworkLib/PHY//MAC Transceiver/Subsystem/BusSwitchFunOut/1to2_3 ==
  In : Inport
  C : Inport  Port=2
  Logical Operator1 : Logic  AllPortsSameDT=off  OutDataTypeStr=boolean
  Logical Operator2 : Logic  AllPortsSameDT=off  OutDataTypeStr=boolean
  Logical Operator3 : Logic  Operator=NOT  AllPortsSameDT=off  OutDataTypeStr=boolean
  Out1 : Outport  VectorParamsAs1DForOutWhenUnconnected=off
  Out2 : Outport  Port=2  VectorParamsAs1DForOutWhenUnconnected=off
  wires:
  Logical Operator2/1 -> Out2/1
  C/1 -> Logical Operator1/2, Logical Operator3/1
  In/1 -> Logical Operator2/1, Logical Operator1/1
  Logical Operator1/1 -> Out1/1
  Logical Operator3/1 -> Logical Operator2/2

== system PacketizedNetworkLib/PHY//MAC Transceiver/Subsystem/BusSwitchFunOut/1to2_5 ==
  In : Inport
  C : Inport  Port=2
  Logical Operator1 : Logic  AllPortsSameDT=off  OutDataTypeStr=boolean
  Logical Operator2 : Logic  AllPortsSameDT=off  OutDataTypeStr=boolean
  Logical Operator3 : Logic  Operator=NOT  AllPortsSameDT=off  OutDataTypeStr=boolean
  Out1 : Outport  VectorParamsAs1DForOutWhenUnconnected=off
  Out2 : Outport  Port=2  VectorParamsAs1DForOutWhenUnconnected=off
  wires:
  Logical Operator2/1 -> Out2/1
  C/1 -> Logical Operator1/2, Logical Operator3/1
  In/1 -> Logical Operator2/1, Logical Operator1/1
  Logical Operator1/1 -> Out1/1
  Logical Operator3/1 -> Logical Operator2/2

== system PacketizedNetworkLib/PHY//MAC Transceiver/Subsystem/BusSwitchFunOut/1to2_6 ==
  In : Inport
  C : Inport  Port=2
  Logical Operator1 : Logic  AllPortsSameDT=off  OutDataTypeStr=boolean
  Logical Operator2 : Logic  AllPortsSameDT=off  OutDataTypeStr=boolean
  Logical Operator3 : Logic  Operator=NOT  AllPortsSameDT=off  OutDataTypeStr=boolean
  Out1 : Outport  VectorParamsAs1DForOutWhenUnconnected=off
  Out2 : Outport  Port=2  VectorParamsAs1DForOutWhenUnconnected=off
  wires:
  Logical Operator3/1 -> Logical Operator2/2
  Logical Operator1/1 -> Out1/1
  In/1 -> Logical Operator1/1, Logical Operator2/1
  C/1 -> Logical Operator3/1, Logical Operator1/2
  Logical Operator2/1 -> Out2/1

== system PacketizedNetworkLib/PHY//MAC Transceiver/Subsystem/BusSwitchFunOut/1to2_Integer ==
  In : Inport
  C : Inport  Port=2
  Constant : Constant  Value=0  OutDataTypeStr=int16  SampleTime=-1
  Logical Operator3 : Logic  Operator=NOT  AllPortsSameDT=off  OutDataTypeStr=boolean
  Switch : Switch  Criteria=u2 > Threshold  SaturateOnIntegerOverflow=off  InputSameDT=off
  Switch1 : Switch  Criteria=u2 > Threshold  SaturateOnIntegerOverflow=off  InputSameDT=off
  Out1 : Outport  VectorParamsAs1DForOutWhenUnconnected=off
  Out2 : Outport  Port=2  VectorParamsAs1DForOutWhenUnconnected=off
  wires:
  Logical Operator3/1 -> Switch1/2
  Switch/1 -> Out1/1
  C/1 -> Switch/2, Logical Operator3/1
  Switch1/1 -> Out2/1
  Constant/1 -> Switch/3, Switch1/3
  In/1 -> Switch1/1, Switch/1

== matlab function PacketizedNetworkLib/DFE/Sign_C  ==
  data: u input; y output
function y = fcn(u)
y=0.707*complex(sign(real(u)), sign(imag(u)));

== stateflow chart PacketizedNetworkLib/Demodulator and CRC/PyldLngth Gen ==
  settings: executeAtInitialization=1
  state RxStandby
  state HerderErr
    en:
    K=K-1;
    RxErr=1;
  state HeaderOn
    en:
    RxLngth=RxLngth+bitshift(int16(RxIn), 16-i);
    i=i+1;
  state PyldCntrl
    en:
    RxCrc=logical(1);
    RxLngth=RxLngth-1;
  note: Indentify Payload Length
  (default) -> (junction 31)
  PyldCntrl -> (junction 31) [order 1] : [RxLngth<=0]
      | {RxCrc=logical(0);}
  HerderErr -> (junction 31) [order 1] : [K==0]
      | {RxErr=0;}
  (junction 51) -> (junction 31) [order 1] : [RxLngth<=0]
  HeaderOn -> (junction 31) [order 4] : [i>16]
  (junction 31) -> RxStandby
  RxStandby -> HeaderOn : [Start==1]
      | {i=1;
      | RxLngth=0;
      | RxCrc=logical(0);
      | RxBits=logical(0);}
  HerderErr -> HerderErr [order 2]
  (junction 47) -> PyldCntrl [order 2] : {RxBits=logical(1);}
  (junction 47) -> PyldCntrl [order 1] : [RxLngth<=32]
      | {RxBits=logical(0);}
  PyldCntrl -> (junction 47) [order 2]
  HeaderOn -> HerderErr [order 2] : [Err==1]
      | {K=16;}
  HeaderOn -> (junction 51) [order 1] : [End==1 && Err==0]
  (junction 51) -> PyldCntrl [order 2] : {RxBits=logical(1);}
  HeaderOn -> HeaderOn [order 3] : [i<=16]
  data: RxIn input; Start input; Err input; End input; RxCrc output boolean; i local int16; RxLngth local int16; K local; RxBits output boolean; RxErr output

== stateflow chart PacketizedNetworkLib/Demodulator and CRC/RxType Gen ==
  settings: executeAtInitialization=1
  state Delay
    en:
    K=K-1;
  state RxData
    en:
    RxDataOk=logical(1);
  state RxAck
    en:
    RxAckOk=logical(1);
  state Delay1
    en:
    RxErr=logical(1);
  state DropPacket
  state RxStandby
  state RxOp
    en: RxHold=1;
  state ToAddGen
    en: RxToAdd(Kbp-7)=RxIn;
  note: Note: Parameter NodeAddre contains the node address:
      |           Node1 is 01, Node2 is 10, and Node3 is 11
  state DataTypeGen
  note: Identify Packet Type and To Address
  Delay -> Delay [order 2]
  (default) -> (junction 31)
  (junction 67) -> Delay : {K=16;}
  Delay -> (junction 31) [order 1] : [K==0]
  RxData -> (junction 67) : {RxDataOn=logical(0);}
  RxAck -> (junction 67)
  (junction 39) -> RxAck [order 2] : [sum(TypeAck,'native')==0]
  (junction 39) -> RxData [order 1] : [sum(TypeData,'native')==0]
  (junction 31) -> RxStandby : {RxType=zeros(1,4);
      | RxToAdd=zeros(1,8);
      | RxDataOk=logical(0);
      | RxDataOn=logical(0);
      | RxAckOk=logical(0);
      | RxHold=0;
      | RxErr=logical(0);}
  Delay1 -> (junction 31)
  RxOp -> (junction 31) : {RxHold=0;}
  DropPacket -> (junction 39) [order 2] : [End==1&&Err==0]
  DropPacket -> Delay1 [order 1] : [Err==1]
  (junction 99) -> DropPacket [order 2]
  (junction 99) -> DropPacket [order 1] : [sum(TypeData,'native')==0]
      | {RxDataOn=logical(1);}
  RxStandby -> DataTypeGen : [Start==1]
      | {Kbp=1;
      | RxType(Kbp)=RxIn;}
  (junction 75) -> (junction 99) [order 1] : [sum(AddCom,'native')==0]
  (junction 75) -> RxOp [order 2]
  ToAddGen -> (junction 75) [order 1] : [Kbp==15]
      | {AddCom=bitxor(RxToAdd, int8(NodeAddre));}
  DataTypeGen -> DataTypeGen [order 1] : [Kbp<4]
      | {Kbp=Kbp+1;
      | RxType(Kbp)=RxIn;}
  DataTypeGen -> ToAddGen [order 2] : [Kbp==8]
      | {TypeData=bitxor(RxType, int8([0 0 1 1]));
      |  TypeAck=bitxor(RxType, int8([1 1 0 0]));}
  DataTypeGen -> DataTypeGen [order 3] : {Kbp=Kbp+1;}
  ToAddGen -> ToAddGen [order 2] : [Kbp<15]
      | {Kbp=Kbp+1;}
  data: RxIn input; Start input; Err input; End input; Kbp local int8; RxDataOk output boolean; RxAckOk output boolean; RxType local int8; K local int16; RxToAdd local int8; RxHold local int8; TypeData local int8; TypeAck local int8; AddCom local int8; RxDataOn output boolean; RxErr output; NodeAddre parameter

== stateflow chart PacketizedNetworkLib/PHY//MAC Transceiver/Subsystem/ALOHA MAC Layer ==
  state Delay
  state Reset
  state Tx1 DATA [group]
    state Reset1
    state AckWait
      en:
      AckWaitTime=AckWaitTime-1;
    state TxOn
      en:
      TxTime=TxTime-1;
      TxDataOn=1;
    state Delay2
      en:
      TxK=TxK-1;
    state TurnOnTxSw
      en:
      TxDataSIFS=TxDataSIFS-1;
      TxSwOn=1;
    state Backoff
      en:
      BOTime=BOTime-1;
    Reset1 -> (junction 327)
    (junction 327) -> TurnOnTxSw [order 1] : [TxEn==1]
        | {CW=15;
        | BONum=0;
        | TxDataDone=0;
        | TxTime=TxLength;
        | TxDataSIFS=SIFS;}
    AckWait -> Reset1 [order 1] : [AckOk==1&&AckWaitTime>0]
        | {TxDataDone=1;}
    TurnOnTxSw -> TxOn [order 1] : [TxDataSIFS<=0]
    TxOn -> Delay2 [order 1] : [TxTime==0]
        | {AckWaitTime=AckLength+64;
        | TxDataOn=0;
        | TxK=2;}
    Delay2 -> AckWait [order 1] : [TxK==0]
        | {TxSwOn=0;}
    Delay2 -> Delay2 [order 2]
    TurnOnTxSw -> TurnOnTxSw [order 2]
    Backoff -> TurnOnTxSw [order 3] : [BOTime<=0]
        | {BONum=BONum+1;
        | TxTime=TxLength;}
    TxOn -> TxOn [order 2] : [TxTime>0]
    AckWait -> AckWait [order 3] : [AckWaitTime>0]
    (junction 354) -> Backoff [order 1] : [BONum==0]
        | {BOTime=randi([0 CW],1)*SLOT;}
    (junction 354) -> Backoff [order 2] : {CW=CW*2+1;
        |  BOTime=randi([0 CW],1)*SLOT;}
    Backoff -> Backoff [order 2] : [BOTime>0]
  state StandBy
  state Tx ACK [group]
    state Delay1
      en:
      TxK=TxK-1;
    state RxDataOK
      en:
      TxAckSIFS=TxAckSIFS-1;
      TxSwOn=1;
    state AckOn
      en:
      TxAckTime=TxAckTime-1;
      TxAckOn=1;
      TxSwOn=1;
    (junction 394) -> RxDataOK : {TxAckSIFS=SIFS;}
    Delay1 -> Delay1 [order 2]
    AckOn -> Delay1 [order 1] : [TxAckTime==0]
        | {TxAckOn=0;
        | TxK=2;}
    RxDataOK -> AckOn [order 1] : [TxAckSIFS<=0]
        | {TxAckTime=AckLength;}
    RxDataOK -> RxDataOK [order 2]
    AckOn -> AckOn [order 2]
  note: Note: The MAC time unit is 8 times the symbol time (Ts), or 16 times the bit time.
      |           TxLength: data packet bit length divided by 16 = 529*(8000+464)/16.
      |   	    SLOT: backoff duration = TxLength/2.  With carrier sense or NAV, SLOT can be much smaller.
      |              In 802.11, SLOT is 20 us (5us turn around and 15us energy detection)
      |           CW: contention window length (number of SLOTs).
      | 	    BOTime: random back off time = randi([0 CW],1)*SLOT;
      |           SIFS: short interframe spacing is the idle time between the end of a data packet and the start of the ACK packet. It is set to 2 MAC time units (= 2x16 bits).
      |           AckLength: ack duration in MAC time units (number of ACK bits / 16)
      |           AckWaitTime: timer for AckWait state
      |           BoNum: number of backoff attempts.
      |
      |           AckOK: status of ACK packet CRC.
      |
      |           TxDataDone: output to LLC sublayer indicating that the current packet is transmitted OK.
      |           TxDataFail: output to LLC sublayer indicating that the current packet has failed.
  (default) -> (junction 372) : {
      | SLOT=floor(TxLength/2);     %SLOT time
      | SIFS=2;                        % Tx/Rx Turnaround
      | AckLength=400/16;      %Ack length = 400 bits, here "16" is the number of bits for MAC step size in bits
      | CWmax=31;
      | rng(pseed);
      | TxDataFail=0;
      | TxDataDone=0;
      | BONum=0;
      | SigD=0;       % Signal detection is set to zero for the case that the carrier sense is not used
      | }
  (junction 374) -> Delay
  Reset -> (junction 374) : {TxDataFail=0;}
  Delay -> (junction 372)
  (junction 327) -> (junction 374) [order 2] : {TxDataDone=0;}
  (junction 372) -> StandBy : {CW=15;
      | BONum=0;
      | BOTime=0;}
  (junction 330) -> Reset [order 2] : [CW==CWmax]
      | {TxDataFail=1;}
  AckWait -> (junction 330) [order 2] : [AckWaitTime==0]
  StandBy -> TurnOnTxSw [order 2] : [TxEn==1&&SigD==0]
      | {TxTime=TxLength;
      | TxDataSIFS=SIFS;}
  (junction 330) -> (junction 354) [order 1] : [CW<CWmax]
  (junction 434) -> StandBy [order 2]
  (junction 434) -> Backoff [order 1] : [BOTime>0]
  Delay1 -> (junction 434) [order 1] : [TxK==0]
      | {TxSwOn=0;}
  StandBy -> (junction 394) [order 1] : [RxDataOk==1]
  Backoff -> (junction 394) [order 1] : [RxDataOk==1]
  data: TxLength input double; TxEn input; RxDataOk input; AckOk input; TxDataFail output double; TxDataDone output double; AckLength local double; BONum local double; SIFS local double; CWmax local double; CW local double; SLOT local double; TxTime local double; TxDataOn output double; SigD local; TxK local; TxAckOn output; BOTime output double; AckWaitTime output double; TxAckTime local; TxDataSIFS local; TxAckSIFS local; TxSwOn local; pseed parameter
